simulink library "casper_library_communications"  (Simulink 8.0)
settings: Solver=ode45  SolverMode=SingleTasking  StartTime=0.0  StopTime=10.0  RelTol=1e-3
undefined symbols (not defined in the file or in its folder): Down, Up
libraries: xbsIndex_r4 x340, xbsReplacements_r4 x6, xps_library x2, casper_library_misc x1
(part 2 of 2)

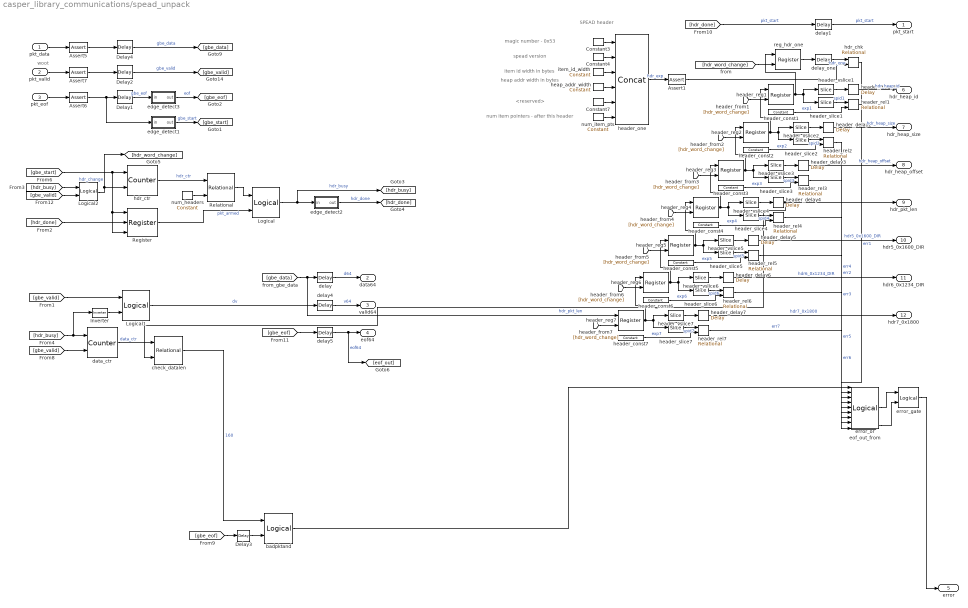
== system casper_library_communications/spead_unpack ==
  note: num item pointers -
      | after this header
  note: <reserved>
  note: heap addr width in bytes
  note: item id width in bytes
  note: spead version
  note: magic number - 0x53
  note: SPEAD header
  note: woot
  pkt_data : Inport
  pkt_valid : Inport  Port=2
  pkt_eof : Inport  Port=3
  Assert1 : xbsIndex_r4/Assert  assert_type=on  type_source=Explicitly  gui_display_data_type=Fixed-point  arith_type=Unsigned  n_bits=64  bin_pt=0  preci_type=Single  exp_width=8  frac_width=24  assert_rate=off  rate_source=Explicitly  period=1  output_port=on  block_type=assert
      settings: block_version=10.1.3
  Assert5 : xbsIndex_r4/Assert  assert_type=on  type_source=Explicitly  gui_display_data_type=Fixed-point  arith_type=Unsigned  n_bits=64  bin_pt=0  preci_type=Single  exp_width=8  frac_width=24  assert_rate=off  rate_source=Explicitly  period=1  output_port=on  block_type=assert
      settings: block_version=10.1.3
  Assert6 : xbsIndex_r4/Assert  assert_type=on  type_source=Explicitly  gui_display_data_type=Boolean  arith_type=Boolean  n_bits=spead_msw  bin_pt=0  preci_type=Single  exp_width=8  frac_width=24  assert_rate=off  rate_source=Explicitly  period=1  output_port=on  block_type=assert
      settings: block_version=10.1.3
  Assert7 : xbsIndex_r4/Assert  assert_type=on  type_source=Explicitly  gui_display_data_type=Boolean  arith_type=Boolean  n_bits=64  bin_pt=0  preci_type=Single  exp_width=8  frac_width=24  assert_rate=off  rate_source=Explicitly  period=1  output_port=on  block_type=assert
      settings: block_version=10.1.3
  Constant3 : xbsIndex_r4/Constant  const=83  gui_display_data_type=Fixed-point  arith_type=Unsigned  n_bits=8  bin_pt=0  preci_type=Single  exp_width=8  frac_width=24  explicit_period=on  period=1  equ=P=C  opselect=C  inp2=PCIN>>17  opr=+  inp1=P  carry=CIN  dbl_ovrd=off  block_type=constant
  Constant4 : xbsIndex_r4/Constant  const=spead_version  gui_display_data_type=Fixed-point  arith_type=Unsigned  n_bits=8  bin_pt=0  preci_type=Single  exp_width=8  frac_width=24  explicit_period=on  period=1  equ=P=C  opselect=C  inp2=PCIN>>17  opr=+  inp1=P  carry=CIN  dbl_ovrd=off  block_type=constant
  Constant7 : xbsIndex_r4/Constant  const=0  gui_display_data_type=Fixed-point  arith_type=Unsigned  n_bits=16  bin_pt=0  preci_type=Single  exp_width=8  frac_width=24  explicit_period=on  period=1  equ=P=C  opselect=C  inp2=PCIN>>17  opr=+  inp1=P  carry=CIN  dbl_ovrd=off  block_type=constant
  Delay{1..4} (4 alike) : xbsIndex_r4/Delay  rst=off  infoeditControl=Selection of Reset will increase slice count due to use of real FFs and instead of SRLs  en=off  latency=1  dbl_ovrd=off  reg_retiming=on  block_type=delay
      settings: block_version=11.4
  Inverter : xbsIndex_r4/Inverter  en=off  latency=0  dbl_ovrd=off  block_type=inv
  Logical : xbsIndex_r4/Logical  logical_function=AND  inputs=2  en=off  latency=0  precision=Full  arith_type=Unsigned  n_bits=16  bin_pt=0  align_bp=on  dbl_ovrd=off  block_type=logical
  Logical1 : xbsIndex_r4/Logical  logical_function=AND  inputs=2  en=off  latency=0  precision=Full  arith_type=Unsigned  n_bits=16  bin_pt=0  align_bp=on  dbl_ovrd=off  block_type=logical
  Logical2 : xbsIndex_r4/Logical  logical_function=AND  inputs=2  en=off  latency=0  precision=Full  arith_type=Unsigned  n_bits=16  bin_pt=0  align_bp=on  dbl_ovrd=off  block_type=logical
  Register : xbsIndex_r4/Register  init=0  rst=on  en=on  dbl_ovrd=off  block_type=register
  Relational : xbsIndex_r4/Relational  mode=a<b  en=off  latency=0  dbl_ovrd=off  block_type=relational
  badpktand : xbsIndex_r4/Logical  logical_function=AND  inputs=2  en=off  latency=0  precision=Full  arith_type=Unsigned  n_bits=16  bin_pt=0  align_bp=on  dbl_ovrd=off  block_type=logical
  check_datalen : xbsIndex_r4/Relational  mode=a!=b  en=off  latency=0  dbl_ovrd=off  block_type=relational
  data_ctr : xbsIndex_r4/Counter  cnt_type=Free Running  cnt_to=Inf  operation=Up  start_count=0  cnt_by_val=1  arith_type=Unsigned  n_bits=max_pkt_len_bits + 1  bin_pt=0  load_pin=off  rst=on  en=on  explicit_period=on  period=1  dbl_ovrd=off  use_behavioral_HDL=on  implementation=Fabric  block_type=counter
  delay : xbsIndex_r4/Delay  rst=off  infoeditControl=Selection of Reset will increase slice count due to use of real FFs and instead of SRLs  en=off  latency=2  dbl_ovrd=off  reg_retiming=on  block_type=delay
  delay1 : xbsIndex_r4/Delay  rst=off  infoeditControl=Selection of Reset will increase slice count due to use of real FFs and instead of SRLs  en=off  latency=1  dbl_ovrd=off  reg_retiming=on  block_type=delay
  delay4 : xbsIndex_r4/Delay  rst=off  infoeditControl=Selection of Reset will increase slice count due to use of real FFs and instead of SRLs  en=off  latency=2  dbl_ovrd=off  reg_retiming=on  block_type=delay
  delay5 : xbsIndex_r4/Delay  rst=off  infoeditControl=Selection of Reset will increase slice count due to use of real FFs and instead of SRLs  en=off  latency=2  dbl_ovrd=off  reg_retiming=on  block_type=delay
  delay_one : xbsIndex_r4/Delay  rst=off  infoeditControl=Selection of Reset will increase slice count due to use of real FFs and instead of SRLs  en=off  latency=1  dbl_ovrd=off  reg_retiming=on  block_type=delay
  edge_detect1 : Subsystem  AncestorBlock=casper_library_misc/edge_detect  mask(edge_detect){edge=Falling, polarity=Active High, x_in=[0 0.08 0.08 0.16 0.16 0.24 0.24 0.32 0.32 0.4], y_in=[-1 -1  1  1  1  1  1  1  1  1], x_out=[0.6 0.68 0.68 0.76 0.76 0.84 0.84 0.92 0.92 1], y_out=[-1 -1  1  1 -1 -1 -1 -1 -1 -1]}
      mask prompts: edge "Edge Type"; polarity "Output Polarity"; x_in "Input X Positions"; y_in "Input Y Positions"; x_out "Output X Positions"; y_out "Output Y Positions"
      mask help: Output is active for one-cycle after each edge of the specified type (i.e. rising, falling or both).
      mask init: same as casper_library_communications/spead_pack/edge_detect1
      settings: AttributesFormatString=|
      | falling edges
      | active high
      mask Help: Output is active for one-cycle after each edge of the specified type (i.e. rising, falling, or both).  Latency is zero.
      mask TypeOptions edge: Rising | Falling | Both
      mask TypeOptions polarity: Active High | Active Low
      mask Display:
      | plot(x_in_num,0.5+y_in_num*0.2);
      | plot(x_out_num,0.5+y_out_num*0.2);
  edge_detect2 : Subsystem  AncestorBlock=casper_library_misc/edge_detect  mask(edge_detect){edge=Falling, polarity=Active High, x_in=[0 0.08 0.08 0.16 0.16 0.24 0.24 0.32 0.32 0.4], y_in=[-1 -1  1  1  1  1  1  1  1  1], x_out=[0.6 0.68 0.68 0.76 0.76 0.84 0.84 0.92 0.92 1], y_out=[-1 -1  1  1 -1 -1 -1 -1 -1 -1]}
      mask prompts: edge "Edge Type"; polarity "Output Polarity"; x_in "Input X Positions"; y_in "Input Y Positions"; x_out "Output X Positions"; y_out "Output Y Positions"
      mask help: Output is active for one-cycle after each edge of the specified type (i.e. rising, falling or both).
      mask init: same as casper_library_communications/spead_pack/edge_detect1
      settings: AttributesFormatString=|
      | falling edges
      | active high
      mask Help: Output is active for one-cycle after each edge of the specified type (i.e. rising, falling, or both).  Latency is zero.
      mask TypeOptions edge: Rising | Falling | Both
      mask TypeOptions polarity: Active High | Active Low
      mask Display:
      | plot(x_in_num,0.5+y_in_num*0.2);
      | plot(x_out_num,0.5+y_out_num*0.2);
  edge_detect3 : Subsystem  AncestorBlock=casper_library_misc/edge_detect  mask(edge_detect){edge=Rising, polarity=Active High, x_in=[0 0.08 0.08 0.16 0.16 0.24 0.24 0.32 0.32 0.4], y_in=[-1 -1  1  1  1  1  1  1  1  1], x_out=[0.6 0.68 0.68 0.76 0.76 0.84 0.84 0.92 0.92 1], y_out=[-1 -1  1  1 -1 -1 -1 -1 -1 -1]}
      mask prompts: edge "Edge Type"; polarity "Output Polarity"; x_in "Input X Positions"; y_in "Input Y Positions"; x_out "Output X Positions"; y_out "Output Y Positions"
      mask help: Output is active for one-cycle after each edge of the specified type (i.e. rising, falling or both).
      mask init: same as casper_library_communications/spead_pack/edge_detect1
      settings: AttributesFormatString=|
      | rising edges
      | active high
      mask Help: Output is active for one-cycle after each edge of the specified type (i.e. rising, falling, or both).  Latency is zero.
      mask TypeOptions edge: Rising | Falling | Both
      mask TypeOptions polarity: Active High | Active Low
      mask Display:
      | plot(x_in_num,0.5+y_in_num*0.2);
      | plot(x_out_num,0.5+y_out_num*0.2);
  error_gate : xbsIndex_r4/Logical  logical_function=AND  inputs=2  en=off  latency=0  precision=Full  arith_type=Unsigned  n_bits=16  bin_pt=0  align_bp=on  dbl_ovrd=off  block_type=logical
  error_or : xbsIndex_r4/Logical  logical_function=OR  inputs=9  en=off  latency=0  precision=Full  arith_type=Unsigned  n_bits=16  bin_pt=0  align_bp=on  dbl_ovrd=off  block_type=logical
  hdr_chk : xbsIndex_r4/Relational  mode=a!=b  en=off  latency=1  dbl_ovrd=off  block_type=relational
  hdr_ctr : xbsIndex_r4/Counter  cnt_type=Free Running  cnt_to=Inf  operation=Up  start_count=0  cnt_by_val=1  arith_type=Unsigned  n_bits=4  bin_pt=0  load_pin=off  rst=on  en=on  explicit_period=on  period=1  dbl_ovrd=off  use_behavioral_HDL=on  implementation=Fabric  block_type=counter
  header_const1 : xbsIndex_r4/Constant  const=8388609  gui_display_data_type=Fixed-point  arith_type=Unsigned  n_bits=spead_msw - spead_lsw  bin_pt=0  preci_type=Single  exp_width=8  frac_width=24  explicit_period=off  period=1  equ=P=C  opselect=C  inp2=PCIN>>17  opr=+  inp1=P  carry=CIN  dbl_ovrd=off  block_type=constant
  header_const2 : xbsIndex_r4/Constant  const=8388610  gui_display_data_type=Fixed-point  arith_type=Unsigned  n_bits=spead_msw - spead_lsw  bin_pt=0  preci_type=Single  exp_width=8  frac_width=24  explicit_period=off  period=1  equ=P=C  opselect=C  inp2=PCIN>>17  opr=+  inp1=P  carry=CIN  dbl_ovrd=off  block_type=constant
  header_const3 : xbsIndex_r4/Constant  const=8388611  gui_display_data_type=Fixed-point  arith_type=Unsigned  n_bits=spead_msw - spead_lsw  bin_pt=0  preci_type=Single  exp_width=8  frac_width=24  explicit_period=off  period=1  equ=P=C  opselect=C  inp2=PCIN>>17  opr=+  inp1=P  carry=CIN  dbl_ovrd=off  block_type=constant
  header_const4 : xbsIndex_r4/Constant  const=8388612  gui_display_data_type=Fixed-point  arith_type=Unsigned  n_bits=spead_msw - spead_lsw  bin_pt=0  preci_type=Single  exp_width=8  frac_width=24  explicit_period=off  period=1  equ=P=C  opselect=C  inp2=PCIN>>17  opr=+  inp1=P  carry=CIN  dbl_ovrd=off  block_type=constant
  header_const5 : xbsIndex_r4/Constant  const=8394240  gui_display_data_type=Fixed-point  arith_type=Unsigned  n_bits=spead_msw - spead_lsw  bin_pt=0  preci_type=Single  exp_width=8  frac_width=24  explicit_period=off  period=1  equ=P=C  opselect=C  inp2=PCIN>>17  opr=+  inp1=P  carry=CIN  dbl_ovrd=off  block_type=constant
  header_const6 : xbsIndex_r4/Constant  const=8393268  gui_display_data_type=Fixed-point  arith_type=Unsigned  n_bits=spead_msw - spead_lsw  bin_pt=0  preci_type=Single  exp_width=8  frac_width=24  explicit_period=off  period=1  equ=P=C  opselect=C  inp2=PCIN>>17  opr=+  inp1=P  carry=CIN  dbl_ovrd=off  block_type=constant
  header_const7 : xbsIndex_r4/Constant  const=6144  gui_display_data_type=Fixed-point  arith_type=Unsigned  n_bits=spead_msw - spead_lsw  bin_pt=0  preci_type=Single  exp_width=8  frac_width=24  explicit_period=off  period=1  equ=P=C  opselect=C  inp2=PCIN>>17  opr=+  inp1=P  carry=CIN  dbl_ovrd=off  block_type=constant
  header_delay{1..7} (7 alike) : xbsIndex_r4/Delay  rst=off  infoeditControl=Selection of Reset will increase slice count due to use of real FFs and instead of SRLs  en=off  latency=2  dbl_ovrd=off  reg_retiming=on  block_type=delay
  header_one : xbsIndex_r4/Concat  num_inputs=6  dbl_ovrd=off  block_type=concat
      settings: block_version=10.1.3
  header_reg{1..7} (7 alike) : xbsIndex_r4/Register  init=0  rst=off  en=on  dbl_ovrd=off  block_type=register
  header_rel{1..7} (7 alike) : xbsIndex_r4/Relational  mode=a!=b  en=off  latency=1  dbl_ovrd=off  block_type=relational
  header_slice{1..7} (7 alike) : xbsIndex_r4/Slice  nbits=spead_msw - spead_lsw  boolean_output=off  mode=Upper Bit Location + Width  bit1=0  base1=MSB of Input  bit0=0  base0=LSB of Input  dbl_ovrd=off  block_type=slice
  header_vslice{1..7} (7 alike) : xbsIndex_r4/Slice  nbits=spead_lsw  boolean_output=off  mode=Lower Bit Location + Width  bit1=0  base1=MSB of Input  bit0=0  base0=LSB of Input  dbl_ovrd=off  block_type=slice
  heap_addr_width : xbsIndex_r4/Constant  const=spead_lsw/8  gui_display_data_type=Fixed-point  arith_type=Unsigned  n_bits=8  bin_pt=0  preci_type=Single  exp_width=8  frac_width=24  explicit_period=on  period=1  equ=P=C  opselect=C  inp2=PCIN>>17  opr=+  inp1=P  carry=CIN  dbl_ovrd=off  block_type=constant
  item_id_width : xbsIndex_r4/Constant  const=(spead_msw-spead_lsw)/8  gui_display_data_type=Fixed-point  arith_type=Unsigned  n_bits=8  bin_pt=0  preci_type=Single  exp_width=8  frac_width=24  explicit_period=on  period=1  equ=P=C  opselect=C  inp2=PCIN>>17  opr=+  inp1=P  carry=CIN  dbl_ovrd=off  block_type=constant
  num_headers : xbsIndex_r4/Constant  const=8  gui_display_data_type=Fixed-point  arith_type=Unsigned  n_bits=4  bin_pt=0  preci_type=Single  exp_width=8  frac_width=24  explicit_period=on  period=1  equ=P=C  opselect=C  inp2=PCIN>>17  opr=+  inp1=P  carry=CIN  dbl_ovrd=off  block_type=constant
  num_item_pts : xbsIndex_r4/Constant  const=7  gui_display_data_type=Fixed-point  arith_type=Unsigned  n_bits=16  bin_pt=0  preci_type=Single  exp_width=8  frac_width=24  explicit_period=on  period=1  equ=P=C  opselect=C  inp2=PCIN>>17  opr=+  inp1=P  carry=CIN  dbl_ovrd=off  block_type=constant
  reg_hdr_one : xbsIndex_r4/Register  init=0  rst=off  en=on  dbl_ovrd=off  block_type=register
  pkt_start : Outport
  data64 : Outport  Port=2
  valid64 : Outport  Port=3
  eof64 : Outport  Port=4
  error : Outport  Port=5
  hdr_heap_id : Outport  Port=6
  hdr_heap_size : Outport  Port=7
  hdr_heap_offset : Outport  Port=8
  hdr_pkt_len : Outport  Port=9
  hdr5_0x1600_DIR : Outport  Port=10
  hdr6_0x1234_DIR : Outport  Port=11
  hdr7_0x1800 : Outport  Port=12
  wires:
  delay/1 -> data64/1  "d64"
  Logical1/1 -> delay4/1  "dv"
  delay5/1 -> [eof_out], eof64/1  "eof64"
  delay4/1 -> valid64/1  "v64"
  [gbe_eof] -> delay5/1
  Delay4/1 -> [gbe_data]  "gbe_data"
  Delay2/1 -> [gbe_valid]  "gbe_valid"
  Delay1/1 -> edge_detect3/1(in)  "gbe_eof"
  [gbe_valid] -> Logical2/2
  Logical2/1 -> hdr_ctr/2, [hdr_word_change]  "hdr_change"
  [hdr_busy] -> Logical2/1
  edge_detect3/1(out) -> [gbe_eof]  "eof"
  [gbe_valid] -> Logical1/1
  Inverter/1 -> Logical1/2
  [hdr_done] -> Register/2
  [hdr_done] -> delay1/1  "pkt_start"
  Delay3/1 -> badpktand/2
  [gbe_eof] -> Delay3/1
  data_ctr/1 -> check_datalen/1  "data_ctr"
  [gbe_valid] -> data_ctr/2
  [hdr_busy] -> data_ctr/1, Inverter/1
  [gbe_data] -> delay/1, header_reg7/1
  Logical/1 -> [hdr_busy], edge_detect2/1(in)  "hdr_busy"
  Register/1 -> Logical/2  "pkt_armed"
  edge_detect2/1(out) -> [hdr_done]  "hdr_done"
  Relational/1 -> Logical/1
  num_headers/1 -> Relational/2
  hdr_ctr/1 -> Relational/1  "hdr_ctr"
  [gbe_start] -> hdr_ctr/1, Register/1, Register/3
  Assert6/1 -> edge_detect1/1(in), Delay1/1
  Assert7/1 -> Delay2/1
  Assert5/1 -> Delay4/1
  edge_detect1/1(out) -> [gbe_start]  "gbe_start"
  pkt_eof/1 -> Assert6/1
  pkt_data/1 -> Assert5/1
  pkt_valid/1 -> Assert7/1
  [hdr_word_change] -> reg_hdr_one/2
  reg_hdr_one/1 -> delay_one/1
  header_one/1 -> Assert1/1  "hdr_exp"
  Constant3/1 -> header_one/1
  Constant4/1 -> header_one/2
  item_id_width/1 -> header_one/3
  heap_addr_width/1 -> header_one/4
  Constant7/1 -> header_one/5
  Assert1/1 -> hdr_chk/2
  delay1/1 -> pkt_start/1  "pkt_start"
  num_item_pts/1 -> header_one/6
  delay_one/1 -> hdr_chk/1  "hdr_one"
  check_datalen/1 -> badpktand/1  "160"
  badpktand/1 -> error_or/1
  hdr_chk/1 -> error_or/2
  error_or/1 -> error_gate/1
  [eof_out] -> error_gate/2
  error_gate/1 -> error/1
  header_reg2/1 -> header_slice2/1, header_vslice2/1, header_reg1/1
  header_reg1/1 -> header_slice1/1, header_vslice1/1, reg_hdr_one/1
  [hdr_word_change] -> header_reg1/2
  header_slice1/1 -> header_rel1/1  "spid1"
  header_vslice1/1 -> header_delay1/1
  header_const1/1 -> header_rel1/2  "exp1"
  header_delay1/1 -> hdr_heap_id/1  "hdr_heap_id"
  header_rel1/1 -> error_or/3  "err1"
  header_reg3/1 -> header_slice3/1, header_vslice3/1, header_reg2/1
  [hdr_word_change] -> header_reg2/2
  header_slice2/1 -> header_rel2/1  "spid2"
  header_vslice2/1 -> header_delay2/1
  header_const2/1 -> header_rel2/2  "exp2"
  header_delay2/1 -> hdr_heap_size/1  "hdr_heap_size"
  header_rel2/1 -> error_or/4  "err2"
  header_reg4/1 -> header_slice4/1, header_vslice4/1, header_reg3/1
  [hdr_word_change] -> header_reg3/2
  header_slice3/1 -> header_rel3/1  "spid3"
  header_vslice3/1 -> header_delay3/1
  header_const3/1 -> header_rel3/2  "exp3"
  header_delay3/1 -> hdr_heap_offset/1  "hdr_heap_offset"
  header_rel3/1 -> error_or/5  "err3"
  header_reg5/1 -> header_slice5/1, header_vslice5/1, header_reg4/1
  [hdr_word_change] -> header_reg4/2
  header_slice4/1 -> header_rel4/1  "spid4"
  header_vslice4/1 -> header_delay4/1
  header_const4/1 -> header_rel4/2  "exp4"
  header_delay4/1 -> hdr_pkt_len/1, check_datalen/2  "hdr_pkt_len"
  header_rel4/1 -> error_or/6  "err4"
  header_reg6/1 -> header_slice6/1, header_vslice6/1, header_reg5/1
  [hdr_word_change] -> header_reg5/2
  header_slice5/1 -> header_rel5/1  "spid5"
  header_vslice5/1 -> header_delay5/1
  header_const5/1 -> header_rel5/2  "exp5"
  header_delay5/1 -> hdr5_0x1600_DIR/1  "hdr5_0x1600_DIR"
  header_rel5/1 -> error_or/7  "err5"
  header_reg7/1 -> header_slice7/1, header_vslice7/1, header_reg6/1
  [hdr_word_change] -> header_reg6/2
  header_slice6/1 -> header_rel6/1  "spid6"
  header_vslice6/1 -> header_delay6/1
  header_const6/1 -> header_rel6/2  "exp6"
  header_delay6/1 -> hdr6_0x1234_DIR/1  "hdr6_0x1234_DIR"
  header_rel6/1 -> error_or/8  "err6"
  [hdr_word_change] -> header_reg7/2
  header_slice7/1 -> header_rel7/1  "spid7"
  header_vslice7/1 -> header_delay7/1
  header_const7/1 -> header_rel7/2  "exp7"
  header_delay7/1 -> hdr7_0x1800/1  "hdr7_0x1800"
  header_rel7/1 -> error_or/9  "err7"

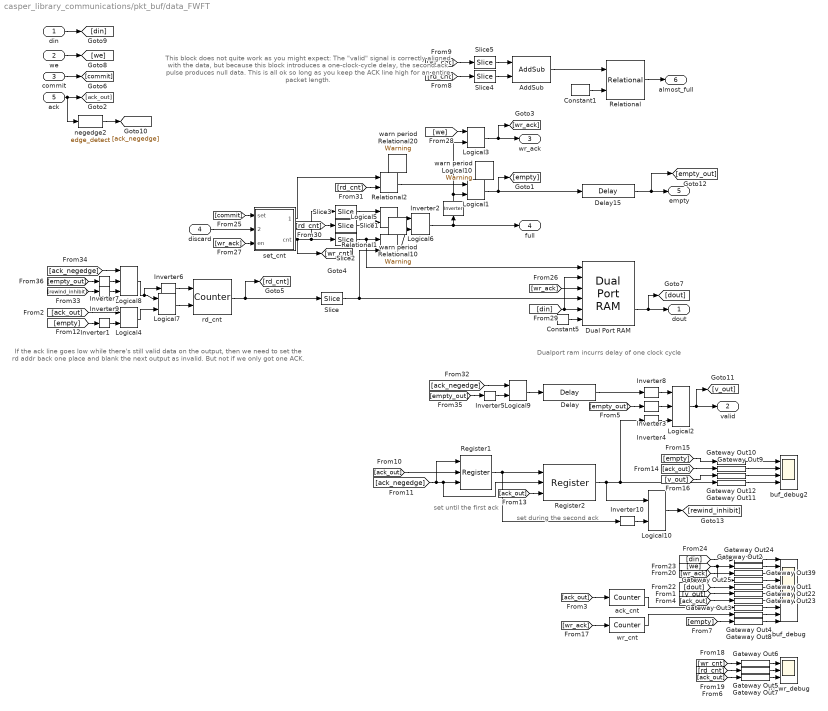
== system casper_library_communications/pkt_buf/data_FWFT ==
  note: Dualport ram incurrs delay
      | of one clock cycle
  note: This block does not quite work as you might expect:
      | The "valid" signal is correctly aligned with the data,
      | but because this block introduces a one-clock-cycle delay,
      | the second ack pulse produces null data.
      |
      | This is all ok so long as you keep the ACK line high for an entire packet length.
  note: If the ack line goes low while there's still valid data on the output,
      | then we need to set the rd addr back one place and blank the next
      | output as invalid. But not if we only got one ACK.
  note: set during the second ack
  note: set until the first ack
  din : Inport
  we : Inport  Port=2
  commit : Inport  Port=3
  discard : Inport  Port=4
  ack : Inport  Port=5
  AddSub : xbsIndex_r4/AddSub  mode=Subtraction  use_carryin=off  use_carryout=off  en=off  latency=0  precision=User Defined  arith_type=Unsigned  n_bits=depth_bits  bin_pt=0  quantization=Truncate  overflow=Wrap  dbl_ovrd=off  use_behavioral_HDL=off  hw_selection=Fabric  pipelined=on  use_rpm=on  block_type=addsub
      settings: block_version=10.1.3
  Constant1 : xbsIndex_r4/Constant  const=(2^depth_bits) - 2^(burst_bits)-1  gui_display_data_type=Fixed-point  arith_type=Unsigned  n_bits=depth_bits+1  bin_pt=0  preci_type=Single  exp_width=8  frac_width=24  explicit_period=on  period=1  equ=P=C  opselect=C  inp2=PCIN>>17  opr=+  inp1=P  carry=CIN  dbl_ovrd=off  block_type=constant
  Constant5 : xbsIndex_r4/Constant  const=0  gui_display_data_type=Fixed-point  arith_type=Boolean  n_bits=1  bin_pt=0  preci_type=Single  exp_width=8  frac_width=24  explicit_period=on  period=1  equ=P=C  opselect=C  inp2=PCIN>>17  opr=+  inp1=P  carry=CIN  dbl_ovrd=off  block_type=constant
  Delay : xbsIndex_r4/Delay  rst=off  infoeditControl=Selection of Reset will increase slice count due to use of real FFs and instead of SRLs  en=off  latency=1  dbl_ovrd=off  reg_retiming=on  block_type=delay
      settings: xl_area=[0, 0, 0, 0, 0, 0, 0]
  Delay15 : xbsIndex_r4/Delay  rst=off  infoeditControl=Selection of Reset will increase slice count due to use of real FFs and instead of SRLs  en=off  latency=1  dbl_ovrd=off  reg_retiming=on  block_type=delay
      settings: xl_area=[0, 0, 0, 0, 0, 0, 0]
  Dual Port RAM : xbsIndex_r4/Dual Port RAM  depth=2^depth_bits  initVector=0  distributed_mem=Block RAM  init_a=0  init_b=0  rst_a=off  rst_b=off  en_a=off  en_b=off  latency=1  write_mode_A=Read Before Write  write_mode_B=Read Before Write  dbl_ovrd=off  optimize=Area  block_type=dpram
      settings: xl_area=[0, 0, 0, 0, 0, 0, 0]  block_version=10.1.3
  Gateway Out{1..12,22..25,39} (17 alike) : xbsIndex_r4/Gateway Out  inherit_from_input=off  hdl_port=on  timing_constraint=None  locs_specified=off  LOCs={}  UseAsDAC=off  DACChannel='1'  block_type=gatewayout
      settings: infoedit="Gateway out block.  Converts Xilinx fixed point inputs into ouputs of type Simulink integer, double, or fixed point.<P><P>Hardware notes:  In hardware these blocks become top level output ports or are discarded, depending on how they are configured."  xl_area=[0, 0, 0, 0, 0, 0, 0]  block_version=10.1.3
  Inverter{1..10} (10 alike) : xbsIndex_r4/Inverter  en=off  latency=0  dbl_ovrd=off  block_type=inv
      settings: xl_area=[0, 0, 0, 0, 0, 0, 0]
  Logical{1,3..4,6,9..10} (6 alike) : xbsIndex_r4/Logical  logical_function=AND  inputs=2  en=off  latency=0  precision=Full  arith_type=Unsigned  n_bits=8  bin_pt=2  align_bp=on  dbl_ovrd=off  block_type=logical
      settings: xl_area=[0, 0, 0, 0, 0, 0, 0]
  Logical2 : xbsIndex_r4/Logical  logical_function=AND  inputs=3  en=off  latency=0  precision=Full  arith_type=Unsigned  n_bits=8  bin_pt=2  align_bp=on  dbl_ovrd=off  block_type=logical
      settings: xl_area=[0, 0, 0, 0, 0, 0, 0]
  Logical5 : xbsIndex_r4/Logical  logical_function=XOR  inputs=2  en=off  latency=0  precision=Full  arith_type=Unsigned  n_bits=8  bin_pt=2  align_bp=on  dbl_ovrd=off  block_type=logical
      settings: xl_area=[0, 0, 0, 0, 0, 0, 0]
  Logical7 : xbsIndex_r4/Logical  logical_function=OR  inputs=2  en=off  latency=0  precision=Full  arith_type=Unsigned  n_bits=8  bin_pt=2  align_bp=on  dbl_ovrd=off  block_type=logical
      settings: xl_area=[0, 0, 0, 0, 0, 0, 0]
  Logical8 : xbsIndex_r4/Logical  logical_function=AND  inputs=3  en=off  latency=0  precision=Full  arith_type=Unsigned  n_bits=8  bin_pt=2  align_bp=on  dbl_ovrd=off  block_type=logical
      settings: xl_area=[0, 0, 0, 0, 0, 0, 0]
  Register1 : xbsIndex_r4/Register  init=0  rst=on  en=on  dbl_ovrd=off  block_type=register
      settings: xl_area=[0, 0, 0, 0, 0, 0, 0]
  Register2 : xbsIndex_r4/Register  init=0  rst=on  en=on  dbl_ovrd=off  block_type=register
      settings: xl_area=[0, 0, 0, 0, 0, 0, 0]
  Relational : xbsIndex_r4/Relational  mode=a>b  en=off  latency=1  dbl_ovrd=off  block_type=relational
      settings: block_version=10.1.3
  Relational1 : xbsIndex_r4/Relational  mode=a=b  en=off  latency=0  dbl_ovrd=off  block_type=relational
      settings: xl_area=[0, 0, 0, 0, 0, 0, 0]  block_version=10.1.3
  Relational2 : xbsIndex_r4/Relational  mode=a=b  en=off  latency=0  dbl_ovrd=off  block_type=relational
      settings: xl_area=[0, 0, 0, 0, 0, 0, 0]  block_version=10.1.3
  Slice{,2,4..5} (4 alike) : xbsIndex_r4/Slice  nbits=1  boolean_output=off  mode=Two Bit Locations  bit1=-1  base1=MSB of Input  bit0=0  base0=LSB of Input  dbl_ovrd=off  block_type=slice
      settings: infoedit="Extracts a given range of bits from each input sample and presents it at the output.  The output type is ordinarily unsigned with binary point at zero, but can be Boolean when the slice is one bit wide.<P><P>Hardware notes: In hardware this block costs nothing."  block_version=10.1.3
  Slice1 : xbsIndex_r4/Slice  nbits=1  boolean_output=on  mode=Upper Bit Location + Width  bit1=0  base1=MSB of Input  bit0=0  base0=LSB of Input  dbl_ovrd=off  block_type=slice
      settings: infoedit="Extracts a given range of bits from each input sample and presents it at the output.  The output type is ordinarily unsigned with binary point at zero, but can be Boolean when the slice is one bit wide.<P><P>Hardware notes: In hardware this block costs nothing."  block_version=10.1.3
  Slice3 : xbsIndex_r4/Slice  nbits=1  boolean_output=on  mode=Upper Bit Location + Width  bit1=0  base1=MSB of Input  bit0=0  base0=LSB of Input  dbl_ovrd=off  block_type=slice
      settings: infoedit="Extracts a given range of bits from each input sample and presents it at the output.  The output type is ordinarily unsigned with binary point at zero, but can be Boolean when the slice is one bit wide.<P><P>Hardware notes: In hardware this block costs nothing."  block_version=10.1.3
  ack_cnt : xbsIndex_r4/Counter  cnt_type=Free Running  cnt_to=Inf  operation=Up  start_count=0  cnt_by_val=1  arith_type=Unsigned  n_bits=depth_bits + 1  bin_pt=0  load_pin=off  rst=off  en=on  explicit_period=on  period=1  dbl_ovrd=off  use_behavioral_HDL=on  implementation=Fabric  use_rpm=on  block_type=counter
      settings: xl_area=[0, 0, 0, 0, 0, 0, 0]
  buf_debug : Scope  NumInputPorts=10
      settings: YMin=12000~0~9500~0~15500~-5~-5~-5~-5~-5  YMax=13300~1~10500~1~17250~5~5~5~5~5  SaveName=ScopeData2
  buf_debug2 : Scope  NumInputPorts=4
      settings: YMin=0~0.95~0~-1  YMax=1~1.05~1~1  SaveName=ScopeData3
  negedge2 : casper_library_misc/edge_detect  edge=Falling  polarity=Active High  x_in=[0 0.08 0.08 0.16 0.16 0.24 0.24 0.32 0.32 0.4]  y_in="[1  1 -1 -1 -1 -1 -1 -1 -1 -1]"  x_out=[0.6 0.68 0.68 0.76 0.76 0.84 0.84 0.92 0.92 1]  y_out="[-1 -1  1  1 -1 -1 -1 -1 -1 -1]"
      settings: AttributesFormatString=|
      | falling edges
      | active high
  rd_cnt : xbsIndex_r4/Counter  cnt_type=Free Running  cnt_to=Inf  operation=Up/Down  start_count=0  cnt_by_val=1  arith_type=Unsigned  n_bits=depth_bits + 1  bin_pt=0  load_pin=off  rst=off  en=on  explicit_period=on  period=1  dbl_ovrd=off  use_behavioral_HDL=on  implementation=Fabric  use_rpm=on  block_type=counter
      settings: xl_area=[0, 0, 0, 0, 0, 0, 0]
  rd_wr_debug : Scope  NumInputPorts=3
      settings: YMin=150~0~0  YMax=300~1~1  SaveName=ScopeData4
  set_cnt : Subsystem
  warn period Logical10 : xbsReplacements_r4/Warning  period=1
  warn period Relational10 : xbsReplacements_r4/Warning  period=1
  warn period Relational20 : xbsReplacements_r4/Warning  period=1
  wr_cnt : xbsIndex_r4/Counter  cnt_type=Free Running  cnt_to=Inf  operation=Up  start_count=0  cnt_by_val=1  arith_type=Unsigned  n_bits=depth_bits + 1  bin_pt=0  load_pin=off  rst=off  en=on  explicit_period=on  period=1  dbl_ovrd=off  use_behavioral_HDL=on  implementation=Fabric  use_rpm=on  block_type=counter
      settings: xl_area=[0, 0, 0, 0, 0, 0, 0]
  dout : Outport
  valid : Outport  Port=2
  wr_ack : Outport  Port=3
  full : Outport  Port=4
  empty : Outport  Port=5
  almost_full : Outport  Port=6
  wires:
  Delay15/1 -> [empty_out], empty/1
  negedge2/1 -> [ack_negedge]
  [rd_cnt] -> Relational2/2
  [rd_cnt] -> Slice1/1
  din/1 -> [din]
  [din] -> Dual Port RAM/5, Dual Port RAM/2
  Logical3/1 -> [wr_ack], wr_ack/1
  [we] -> Logical3/1
  [wr_ack] -> set_cnt/3(en)
  [wr_ack] -> Dual Port RAM/3
  [commit] -> set_cnt/1(set)
  ack/1 -> negedge2/1, [ack_out]
  Logical1/1 -> Delay15/1, [empty]
  Dual Port RAM/2 -> [dout], dout/1
  Constant5/1 -> Dual Port RAM/6
  discard/1 -> set_cnt/2(undo)
  we/1 -> [we]
  Inverter2/1 -> Logical3/2, Logical1/2
  commit/1 -> [commit]
  set_cnt/1(set_cnt) -> Relational2/1
  set_cnt/2(cnt) -> [wr_cnt], Slice2/1, Slice3/1
  Slice/1 -> Dual Port RAM/4, Relational1/2
  Slice2/1 -> Dual Port RAM/1, Relational1/1
  Slice3/1 -> Logical5/1
  Slice1/1 -> Logical5/2
  Relational1/1 -> Logical6/2
  Logical5/1 -> Logical6/1
  Logical6/1 -> full/1, Inverter2/1
  Relational2/1 -> Logical1/1
  Inverter7/1 -> Logical8/2
  [empty_out] -> Inverter7/1
  [ack_negedge] -> Logical8/1
  Logical8/1 -> Logical7/1, Inverter6/1
  Logical4/1 -> Logical7/2
  Logical7/1 -> rd_cnt/2
  Inverter6/1 -> rd_cnt/1
  Inverter1/1 -> Logical4/2
  [ack_out] -> Logical4/1
  [empty] -> Inverter1/1
  rd_cnt/1 -> Slice/1, [rd_cnt]
  Inverter9/1 -> Logical8/3
  [rewind_inhibit] -> Inverter9/1
  [empty_out] -> Inverter3/1
  Inverter8/1 -> Logical2/1
  Inverter4/1 -> Logical2/3
  Delay/1 -> Inverter8/1
  Logical9/1 -> Delay/1
  Inverter5/1 -> Logical9/2
  [empty_out] -> Inverter5/1
  [ack_negedge] -> Logical9/1
  Register2/1 -> Inverter4/1, Gateway Out11/1, Logical10/1
  [din] -> Gateway Out24/1
  [we] -> Gateway Out25/1, Gateway Out2/1
  [dout] -> Gateway Out1/1
  [wr_ack] -> Gateway Out39/1
  [rd_cnt] -> Gateway Out5/1
  [wr_cnt] -> Gateway Out6/1
  [wr_ack] -> wr_cnt/1
  [ack_out] -> Register2/3
  [v_out] -> Gateway Out12/1
  [empty] -> Gateway Out10/1
  [ack_out] -> Gateway Out9/1
  Gateway Out11/1 -> buf_debug2/4
  Gateway Out12/1 -> buf_debug2/3
  Gateway Out9/1 -> buf_debug2/2
  Gateway Out10/1 -> buf_debug2/1
  Register1/1 -> Register2/1, Inverter10/1
  [ack_out] -> Register1/2
  [ack_negedge] -> Register2/2, Register1/3, Register1/1
  Logical2/1 -> [v_out], valid/1
  [empty] -> Gateway Out8/1
  Gateway Out8/1 -> buf_debug/10
  [ack_out] -> Gateway Out7/1
  Gateway Out7/1 -> rd_wr_debug/3
  Gateway Out5/1 -> rd_wr_debug/2
  Gateway Out6/1 -> rd_wr_debug/1
  [ack_out] -> Gateway Out23/1
  [ack_out] -> ack_cnt/1
  [v_out] -> Gateway Out22/1
  wr_cnt/1 -> Gateway Out4/1
  ack_cnt/1 -> Gateway Out3/1
  Gateway Out4/1 -> buf_debug/9
  Gateway Out3/1 -> buf_debug/8
  Gateway Out23/1 -> buf_debug/7
  Gateway Out22/1 -> buf_debug/6
  Gateway Out1/1 -> buf_debug/5
  Gateway Out25/1 -> buf_debug/4
  Gateway Out39/1 -> buf_debug/3
  Gateway Out2/1 -> buf_debug/2
  Gateway Out24/1 -> buf_debug/1
  Inverter10/1 -> Logical10/2
  Logical10/1 -> [rewind_inhibit]
  Inverter3/1 -> Logical2/2
  [rd_cnt] -> Slice4/1
  [wr_cnt] -> Slice5/1
  AddSub/1 -> Relational/1
  Relational/1 -> almost_full/1
  Constant1/1 -> Relational/2
  Slice5/1 -> AddSub/1
  Slice4/1 -> AddSub/2

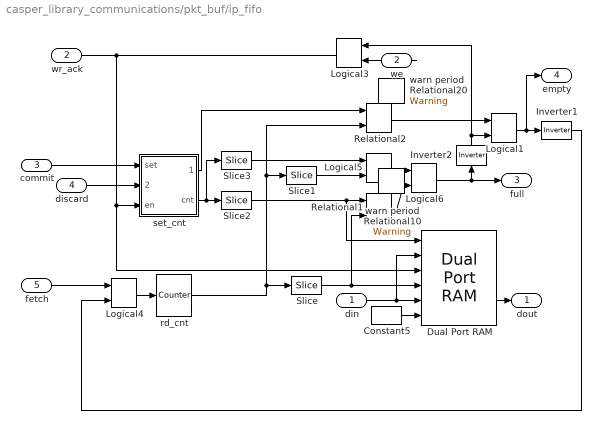
== system casper_library_communications/pkt_buf/ip_fifo ==
  din : Inport
  we : Inport  Port=2
  commit : Inport  Port=3
  discard : Inport  Port=4
  fetch : Inport  Port=5
  Constant5 : xbsIndex_r4/Constant  const=0  gui_display_data_type=Fixed-point  arith_type=Boolean  n_bits=1  bin_pt=0  preci_type=Single  exp_width=8  frac_width=24  explicit_period=on  period=1  equ=P=C  opselect=C  inp2=PCIN>>17  opr=+  inp1=P  carry=CIN  dbl_ovrd=off  block_type=constant
  Dual Port RAM : xbsIndex_r4/Dual Port RAM  depth=2^depth_bits  initVector=0  distributed_mem=Block RAM  init_a=0  init_b=0  rst_a=off  rst_b=off  en_a=off  en_b=off  latency=1  write_mode_A=Read Before Write  write_mode_B=Read Before Write  dbl_ovrd=off  optimize=Area  block_type=dpram
      settings: xl_area=[0, 0, 0, 0, 0, 0, 0]  block_version=10.1.3
  Inverter1 : xbsIndex_r4/Inverter  en=off  latency=0  dbl_ovrd=off  block_type=inv
      settings: xl_area=[0, 0, 0, 0, 0, 0, 0]
  Inverter2 : xbsIndex_r4/Inverter  en=off  latency=0  dbl_ovrd=off  block_type=inv
      settings: xl_area=[0, 0, 0, 0, 0, 0, 0]
  Logical{1,3..4,6} (4 alike) : xbsIndex_r4/Logical  logical_function=AND  inputs=2  en=off  latency=0  precision=Full  arith_type=Unsigned  n_bits=8  bin_pt=2  align_bp=on  dbl_ovrd=off  block_type=logical
      settings: xl_area=[0, 0, 0, 0, 0, 0, 0]
  Logical5 : xbsIndex_r4/Logical  logical_function=XOR  inputs=2  en=off  latency=0  precision=Full  arith_type=Unsigned  n_bits=8  bin_pt=2  align_bp=on  dbl_ovrd=off  block_type=logical
      settings: xl_area=[0, 0, 0, 0, 0, 0, 0]
  Relational1 : xbsIndex_r4/Relational  mode=a=b  en=off  latency=0  dbl_ovrd=off  block_type=relational
      settings: xl_area=[0, 0, 0, 0, 0, 0, 0]  block_version=10.1.3
  Relational2 : xbsIndex_r4/Relational  mode=a=b  en=off  latency=0  dbl_ovrd=off  block_type=relational
      settings: xl_area=[0, 0, 0, 0, 0, 0, 0]  block_version=10.1.3
  Slice : xbsIndex_r4/Slice  nbits=1  boolean_output=off  mode=Two Bit Locations  bit1=-1  base1=MSB of Input  bit0=0  base0=LSB of Input  dbl_ovrd=off  block_type=slice
      settings: infoedit="Extracts a given range of bits from each input sample and presents it at the output.  The output type is ordinarily unsigned with binary point at zero, but can be Boolean when the slice is one bit wide.<P><P>Hardware notes: In hardware this block costs nothing."  block_version=10.1.3
  Slice1 : xbsIndex_r4/Slice  nbits=1  boolean_output=on  mode=Upper Bit Location + Width  bit1=0  base1=MSB of Input  bit0=0  base0=LSB of Input  dbl_ovrd=off  block_type=slice
      settings: infoedit="Extracts a given range of bits from each input sample and presents it at the output.  The output type is ordinarily unsigned with binary point at zero, but can be Boolean when the slice is one bit wide.<P><P>Hardware notes: In hardware this block costs nothing."  block_version=10.1.3
  Slice2 : xbsIndex_r4/Slice  nbits=1  boolean_output=off  mode=Two Bit Locations  bit1=-1  base1=MSB of Input  bit0=0  base0=LSB of Input  dbl_ovrd=off  block_type=slice
      settings: infoedit="Extracts a given range of bits from each input sample and presents it at the output.  The output type is ordinarily unsigned with binary point at zero, but can be Boolean when the slice is one bit wide.<P><P>Hardware notes: In hardware this block costs nothing."  block_version=10.1.3
  Slice3 : xbsIndex_r4/Slice  nbits=1  boolean_output=on  mode=Upper Bit Location + Width  bit1=0  base1=MSB of Input  bit0=0  base0=LSB of Input  dbl_ovrd=off  block_type=slice
      settings: infoedit="Extracts a given range of bits from each input sample and presents it at the output.  The output type is ordinarily unsigned with binary point at zero, but can be Boolean when the slice is one bit wide.<P><P>Hardware notes: In hardware this block costs nothing."  block_version=10.1.3
  rd_cnt : xbsIndex_r4/Counter  cnt_type=Free Running  cnt_to=Inf  operation=Up  start_count=0  cnt_by_val=1  arith_type=Unsigned  n_bits=depth_bits + 1  bin_pt=0  load_pin=off  rst=off  en=on  explicit_period=on  period=1  dbl_ovrd=off  use_behavioral_HDL=on  implementation=Fabric  use_rpm=on  block_type=counter
      settings: xl_area=[0, 0, 0, 0, 0, 0, 0]
  set_cnt : Subsystem
  warn period Relational10 : xbsReplacements_r4/Warning  period=1
  warn period Relational20 : xbsReplacements_r4/Warning  period=1
  dout : Outport
  wr_ack : Outport  Port=2
  full : Outport  Port=3
  empty : Outport  Port=4
  wires:
  Logical4/1 -> rd_cnt/1
  fetch/1 -> Logical4/1
  Inverter1/1 -> Logical4/2
  Logical1/1 -> empty/1, Inverter1/1
  Dual Port RAM/2 -> dout/1
  Constant5/1 -> Dual Port RAM/6
  discard/1 -> set_cnt/2(undo)
  Logical3/1 -> set_cnt/3(en), Dual Port RAM/3, wr_ack/1
  we/1 -> Logical3/2
  Inverter2/1 -> Logical3/1, Logical1/2
  commit/1 -> set_cnt/1(set)
  rd_cnt/1 -> Slice/1, Slice1/1, Relational2/2
  set_cnt/1(set_cnt) -> Relational2/1
  set_cnt/2(cnt) -> Slice3/1, Slice2/1
  Slice/1 -> Dual Port RAM/4, Relational1/2
  din/1 -> Dual Port RAM/5, Dual Port RAM/2
  Slice2/1 -> Dual Port RAM/1, Relational1/1
  Slice3/1 -> Logical5/1
  Slice1/1 -> Logical5/2
  Relational1/1 -> Logical6/2
  Logical5/1 -> Logical6/1
  Logical6/1 -> full/1, Inverter2/1
  Relational2/1 -> Logical1/1

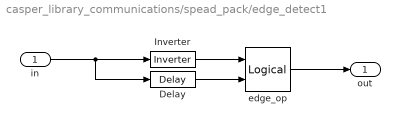
== system casper_library_communications/spead_pack/edge_detect1 ==
  in : Inport
  Delay : xbsIndex_r4/Delay  rst=off  infoeditControl=Selection of Reset will increase slice count due to use of real FFs and instead of SRLs  en=off  latency=1  dbl_ovrd=off  reg_retiming=on  block_type=delay
      settings: xl_area=[0, 0, 0, 0, 0, 0, 0]
  Inverter : xbsIndex_r4/Inverter  en=off  latency=0  dbl_ovrd=off  block_type=inv
      settings: xl_area=[0, 0, 0, 0, 0, 0, 0]
  edge_op : xbsIndex_r4/Logical  logical_function=NOR  inputs=2  en=off  latency=0  precision=Full  arith_type=Unsigned  n_bits=8  bin_pt=2  align_bp=on  dbl_ovrd=off  block_type=logical
      settings: xl_area=[0, 0, 0, 0, 0, 0, 0]
  out : Outport
  wires:
  Inverter/1 -> edge_op/1
  edge_op/1 -> out/1
  in/1 -> Inverter/1, Delay/1
  Delay/1 -> edge_op/2

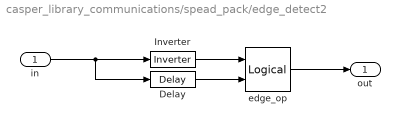
== system casper_library_communications/spead_pack/edge_detect2 ==
  in : Inport
  Delay : xbsIndex_r4/Delay  rst=off  infoeditControl=Selection of Reset will increase slice count due to use of real FFs and instead of SRLs  en=off  latency=1  dbl_ovrd=off  reg_retiming=on  block_type=delay
      settings: xl_area=[0, 0, 0, 0, 0, 0, 0]
  Inverter : xbsIndex_r4/Inverter  en=off  latency=0  dbl_ovrd=off  block_type=inv
      settings: xl_area=[0, 0, 0, 0, 0, 0, 0]
  edge_op : xbsIndex_r4/Logical  logical_function=NOR  inputs=2  en=off  latency=0  precision=Full  arith_type=Unsigned  n_bits=8  bin_pt=2  align_bp=on  dbl_ovrd=off  block_type=logical
      settings: xl_area=[0, 0, 0, 0, 0, 0, 0]
  out : Outport
  wires:
  Delay/1 -> edge_op/2
  in/1 -> Delay/1, Inverter/1
  edge_op/1 -> out/1
  Inverter/1 -> edge_op/1

== system casper_library_communications/spead_unpack/edge_detect1 ==
  in : Inport
  Delay : xbsIndex_r4/Delay  rst=off  infoeditControl=Selection of Reset will increase slice count due to use of real FFs and instead of SRLs  en=off  latency=1  dbl_ovrd=off  reg_retiming=on  block_type=delay
      settings: xl_area=[0, 0, 0, 0, 0, 0, 0]
  Inverter : xbsIndex_r4/Inverter  en=off  latency=0  dbl_ovrd=off  block_type=inv
      settings: xl_area=[0, 0, 0, 0, 0, 0, 0]
  edge_op : xbsIndex_r4/Logical  logical_function=AND  inputs=2  en=off  latency=0  precision=Full  arith_type=Unsigned  n_bits=8  bin_pt=2  align_bp=on  dbl_ovrd=off  block_type=logical
      settings: xl_area=[0, 0, 0, 0, 0, 0, 0]
  out : Outport
  wires:
  Inverter/1 -> edge_op/1
  edge_op/1 -> out/1
  in/1 -> Inverter/1, Delay/1
  Delay/1 -> edge_op/2

== system casper_library_communications/spead_unpack/edge_detect2 ==
  in : Inport
  Delay : xbsIndex_r4/Delay  rst=off  infoeditControl=Selection of Reset will increase slice count due to use of real FFs and instead of SRLs  en=off  latency=1  dbl_ovrd=off  reg_retiming=on  block_type=delay
      settings: xl_area=[0, 0, 0, 0, 0, 0, 0]
  Inverter : xbsIndex_r4/Inverter  en=off  latency=0  dbl_ovrd=off  block_type=inv
      settings: xl_area=[0, 0, 0, 0, 0, 0, 0]
  edge_op : xbsIndex_r4/Logical  logical_function=AND  inputs=2  en=off  latency=0  precision=Full  arith_type=Unsigned  n_bits=8  bin_pt=2  align_bp=on  dbl_ovrd=off  block_type=logical
      settings: xl_area=[0, 0, 0, 0, 0, 0, 0]
  out : Outport
  wires:
  Delay/1 -> edge_op/2
  in/1 -> Delay/1, Inverter/1
  edge_op/1 -> out/1
  Inverter/1 -> edge_op/1

== system casper_library_communications/spead_unpack/edge_detect3 ==
  in : Inport
  Delay : xbsIndex_r4/Delay  rst=off  infoeditControl=Selection of Reset will increase slice count due to use of real FFs and instead of SRLs  en=off  latency=1  dbl_ovrd=off  reg_retiming=on  block_type=delay
      settings: xl_area=[0, 0, 0, 0, 0, 0, 0]
  Inverter : xbsIndex_r4/Inverter  en=off  latency=0  dbl_ovrd=off  block_type=inv
      settings: xl_area=[0, 0, 0, 0, 0, 0, 0]
  edge_op : xbsIndex_r4/Logical  logical_function=NOR  inputs=2  en=off  latency=0  precision=Full  arith_type=Unsigned  n_bits=8  bin_pt=2  align_bp=on  dbl_ovrd=off  block_type=logical
      settings: xl_area=[0, 0, 0, 0, 0, 0, 0]
  out : Outport
  wires:
  Delay/1 -> edge_op/2
  in/1 -> Delay/1, Inverter/1
  edge_op/1 -> out/1
  Inverter/1 -> edge_op/1

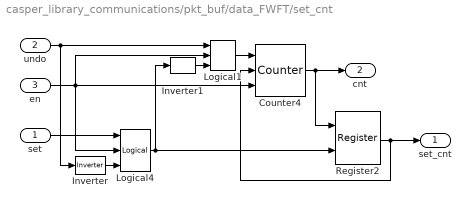
== system casper_library_communications/pkt_buf/data_FWFT/set_cnt ==
  set : Inport
  undo : Inport  Port=2
  en : Inport  Port=3
  Counter4 : xbsIndex_r4/Counter  cnt_type=Free Running  cnt_to=Inf  operation=Up  start_count=0  cnt_by_val=1  arith_type=Unsigned  n_bits=depth_bits + 1  bin_pt=0  load_pin=on  rst=off  en=on  explicit_period=on  period=1  dbl_ovrd=off  use_behavioral_HDL=on  implementation=Fabric  use_rpm=on  block_type=counter
      settings: xl_area=[0, 0, 0, 0, 0, 0, 0]
  Inverter : xbsIndex_r4/Inverter  en=off  latency=0  dbl_ovrd=off  block_type=inv
      settings: xl_area=[0, 0, 0, 0, 0, 0, 0]
  Inverter1 : xbsIndex_r4/Inverter  en=off  latency=0  dbl_ovrd=off  block_type=inv
      settings: xl_area=[0, 0, 0, 0, 0, 0, 0]
  Logical1 : xbsIndex_r4/Logical  logical_function=AND  inputs=3  en=off  latency=0  precision=Full  arith_type=Unsigned  n_bits=8  bin_pt=2  align_bp=on  dbl_ovrd=off  block_type=logical
      settings: xl_area=[0, 0, 0, 0, 0, 0, 0]
  Logical4 : xbsIndex_r4/Logical  logical_function=AND  inputs=3  en=off  latency=1  precision=Full  arith_type=Unsigned  n_bits=8  bin_pt=2  align_bp=on  dbl_ovrd=off  block_type=logical
      settings: xl_area=[0, 0, 0, 0, 0, 0, 0]
  Register2 : xbsIndex_r4/Register  init=0  rst=off  en=on  dbl_ovrd=off  block_type=register
      settings: xl_area=[0, 0, 0, 0, 0, 0, 0]
  set_cnt : Outport
  cnt : Outport  Port=2
  wires:
  Counter4/1 -> cnt/1, Register2/1
  en/1 -> Counter4/3, Logical1/2, Logical4/2
  Register2/1 -> Counter4/2, set_cnt/1
  Logical4/1 -> Register2/2, Inverter1/1
  set/1 -> Logical4/1
  Logical1/1 -> Counter4/1
  undo/1 -> Logical1/1, Inverter/1
  Inverter/1 -> Logical4/3
  Inverter1/1 -> Logical1/3

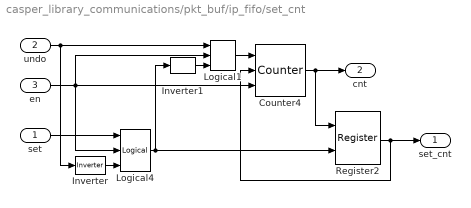
== system casper_library_communications/pkt_buf/ip_fifo/set_cnt ==
  set : Inport
  undo : Inport  Port=2
  en : Inport  Port=3
  Counter4 : xbsIndex_r4/Counter  cnt_type=Free Running  cnt_to=Inf  operation=Up  start_count=0  cnt_by_val=1  arith_type=Unsigned  n_bits=depth_bits + 1  bin_pt=0  load_pin=on  rst=off  en=on  explicit_period=on  period=1  dbl_ovrd=off  use_behavioral_HDL=on  implementation=Fabric  use_rpm=on  block_type=counter
      settings: xl_area=[0, 0, 0, 0, 0, 0, 0]
  Inverter : xbsIndex_r4/Inverter  en=off  latency=0  dbl_ovrd=off  block_type=inv
      settings: xl_area=[0, 0, 0, 0, 0, 0, 0]
  Inverter1 : xbsIndex_r4/Inverter  en=off  latency=0  dbl_ovrd=off  block_type=inv
      settings: xl_area=[0, 0, 0, 0, 0, 0, 0]
  Logical1 : xbsIndex_r4/Logical  logical_function=AND  inputs=3  en=off  latency=0  precision=Full  arith_type=Unsigned  n_bits=8  bin_pt=2  align_bp=on  dbl_ovrd=off  block_type=logical
      settings: xl_area=[0, 0, 0, 0, 0, 0, 0]
  Logical4 : xbsIndex_r4/Logical  logical_function=AND  inputs=3  en=off  latency=1  precision=Full  arith_type=Unsigned  n_bits=8  bin_pt=2  align_bp=on  dbl_ovrd=off  block_type=logical
      settings: xl_area=[0, 0, 0, 0, 0, 0, 0]
  Register2 : xbsIndex_r4/Register  init=0  rst=off  en=on  dbl_ovrd=off  block_type=register
      settings: xl_area=[0, 0, 0, 0, 0, 0, 0]
  set_cnt : Outport
  cnt : Outport  Port=2
  wires:
  Counter4/1 -> cnt/1, Register2/1
  en/1 -> Counter4/3, Logical1/2, Logical4/2
  Register2/1 -> Counter4/2, set_cnt/1
  Logical4/1 -> Register2/2, Inverter1/1
  set/1 -> Logical4/1
  Logical1/1 -> Counter4/1
  undo/1 -> Logical1/1, Inverter/1
  Inverter/1 -> Logical4/3
  Inverter1/1 -> Logical1/3
